simulink model "test1"  (R2025b)
settings: Solver=VariableStepAuto  StartTime=0.0  StopTime=10.0  RelTol=1e-3
values from neighbouring files (symbols this model uses):
  B = 5    [para.m]
  De = 50    [para.m]
  Fc0 = 2    [para.m]
  G = 1    [para.m]
  Ke = 5000    [para.m]
  Kt = 1    [para.m]
  M = 1    [para.m]
  Ti = 0.002    [para.m]
  veps = 0.001    [para.m]
libraries: simulink x2
settings Model: Creator=HYB  LastModifiedBy=HYB

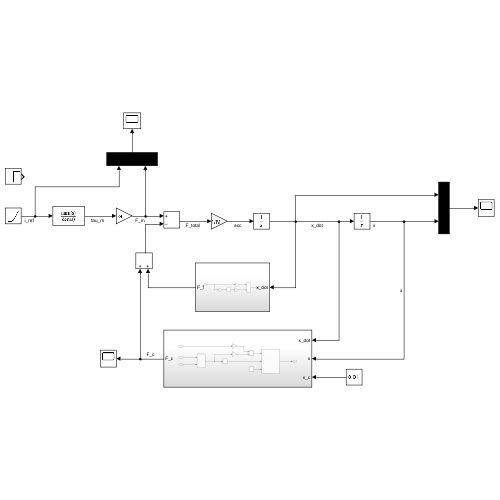
[thumbnail: Simulink's stored preview of the top-level diagram]
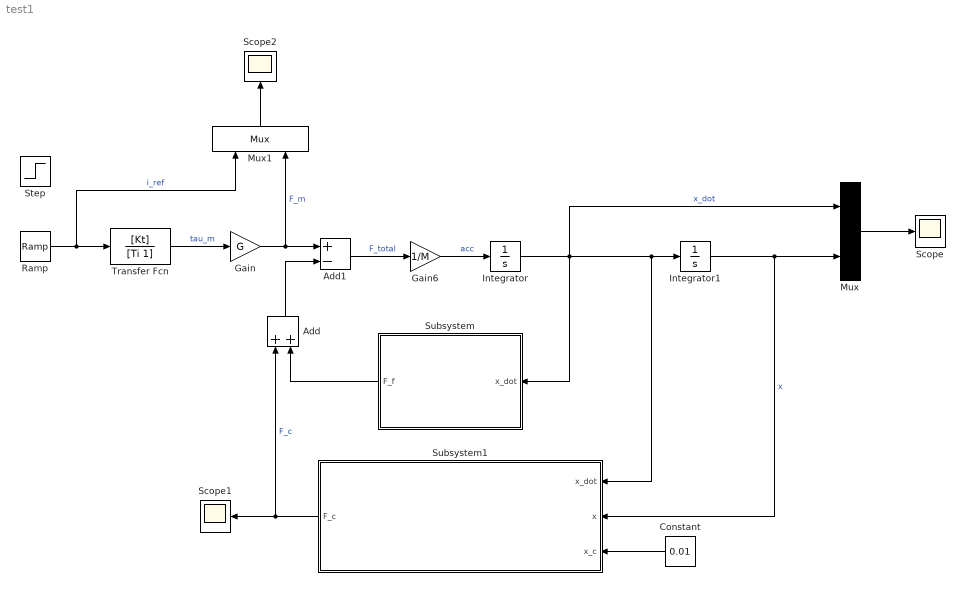
== system test1 ==
  Add : Sum
  Add1 : Sum  Inputs=+-
  Constant : Constant  Value=0.01
  Gain : Gain  Gain=G
  Gain6 : Gain  Gain=1/M
  Integrator : Integrator
  Integrator1 : Integrator
  Mux : Mux  Inputs=2
  Mux1 : Mux  Inputs=2
  Ramp : simulink/Sources/Ramp  slope=10  start=0  InitialOutput=0
  Scope : Scope
      settings: ActiveDisplayYMinimum=-0.026349543052948947  ActiveDisplayYMaximum=0.15768099075861267
  Scope1 : Scope
      settings: ActiveDisplayYMinimum=-23.450299653599771  ActiveDisplayYMaximum=111.66375183013083
  Scope2 : Scope
      settings: ActiveDisplayYMinimum=-12.499999999999996  ActiveDisplayYMaximum=112.5  DataLoggingVariableName=ScopeData2
  Step : Step  SampleTime=0
  Subsystem : Subsystem
  Subsystem1 : Subsystem
  Transfer Fcn : TransferFcn  Numerator=[Kt]  Denominator=[Ti 1]
  wires:
  Transfer Fcn/1 -> Gain/1  "tau_m"
  Add/1 -> Add1/2
  Ramp/1 -> Mux1/1, Transfer Fcn/1  "i_ref"
  Gain/1 -> Mux1/2, Add1/1  "F_m"
  Add1/1 -> Gain6/1  "F_total"
  Gain6/1 -> Integrator/1  "acc"
  Integrator/1 -> Mux/1, Subsystem/1(x_dot), Subsystem1/1(x_dot), Integrator1/1  "x_dot"
  Integrator1/1 -> Mux/2, Subsystem1/2(x)  "x"
  Subsystem/1(F_f) -> Add/2
  Subsystem1/1(F_c) -> Scope1/1, Add/1  "F_c"
  Mux/1 -> Scope/1
  Mux1/1 -> Scope2/1
  Constant/1 -> Subsystem1/3(x_c)

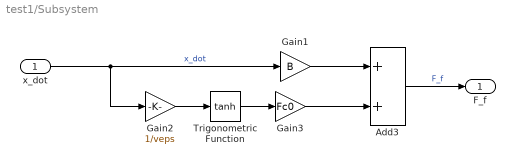
== system test1/Subsystem ==
  x_dot : Inport
  Add3 : Sum
  Gain1 : Gain  Gain=B
  Gain2 : Gain  Gain=1/veps
  Gain3 : Gain  Gain=Fc0
  Trigonometric Function : Trigonometry  Operator=tanh
  F_f : Outport
  wires:
  Trigonometric Function/1 -> Gain3/1
  Add3/1 -> F_f/1  "F_f"
  x_dot/1 -> Gain2/1, Gain1/1  "x_dot"
  Gain3/1 -> Add3/2
  Gain2/1 -> Trigonometric Function/1
  Gain1/1 -> Add3/1

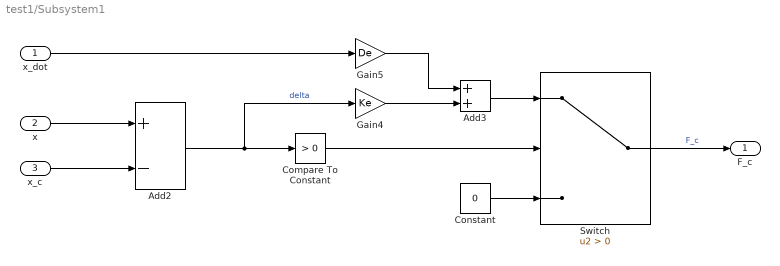
== system test1/Subsystem1 ==
  x_dot : Inport
  x : Inport  Port=2
  x_c : Inport  Port=3
  Add2 : Sum  Inputs=+-
  Add3 : Sum
  Compare To Constant : simulink/Logic and Bit Operations/Compare To Constant  relop=>  const=0  OutDataTypeStr=boolean
  Constant : Constant  Value=0
  Gain4 : Gain  Gain=Ke
  Gain5 : Gain  Gain=De
  Switch : Switch  Criteria=u2 > Threshold  SaturateOnIntegerOverflow=off  InputSameDT=off
  F_c : Outport
  wires:
  x_dot/1 -> Gain5/1
  Add2/1 -> Compare To Constant/1, Gain4/1  "delta"
  x_c/1 -> Add2/2
  x/1 -> Add2/1
  Switch/1 -> F_c/1  "F_c"
  Gain4/1 -> Add3/2
  Gain5/1 -> Add3/1
  Compare To Constant/1 -> Switch/2
  Add3/1 -> Switch/1
  Constant/1 -> Switch/3
